simulink model "quadrotor_lqr_v3"  (R2026a)
settings: Solver=ode4  StopTime=15  FixedStep=1e-3
PreLoadFcn:
  | run('init_params.m'); if exist('controller_data.mat','file'), load('controller_data.mat'); end
values from neighbouring files (symbols this model uses):
  K = [3.16227766017 -4.72567955818e-17 -8.28019285395e-17 -1.64313429263e-16 4.90965597244 1.71076429981e-16 -5.36515533389e-17 3.94835012882e-16 5.96978589095e-16 2.2360679775 -3.44681097997e-15 8.87033425726e-16 ... (32 elements, 4x8)]    [controller_data.mat]    (also in design_lqr.m = lqr(A, B, Q, R))
undefined symbols (not defined in the file or in its folder): ic, params, ref, sat
settings Model: FPTShortcutValueString='{{},{''BaselineRun'',1,1,1,''BaselineRun'','''',{},''M'','''',''''},{''BaselineRun_2'',1,1,1,''BaselineRun_2'','''',{},''M'','''',''''}}'  Creator=yusuf  LastModifiedBy=yusuf

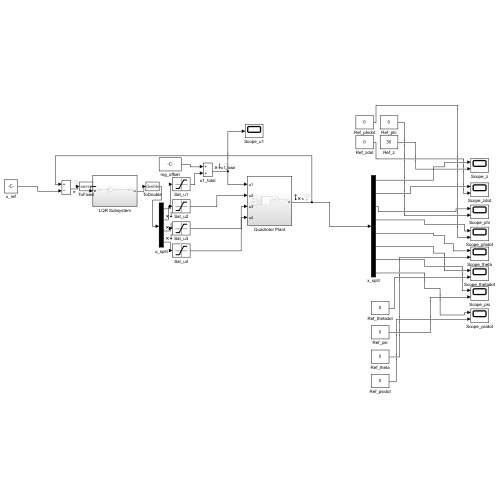
[thumbnail: Simulink's stored preview of the top-level diagram]
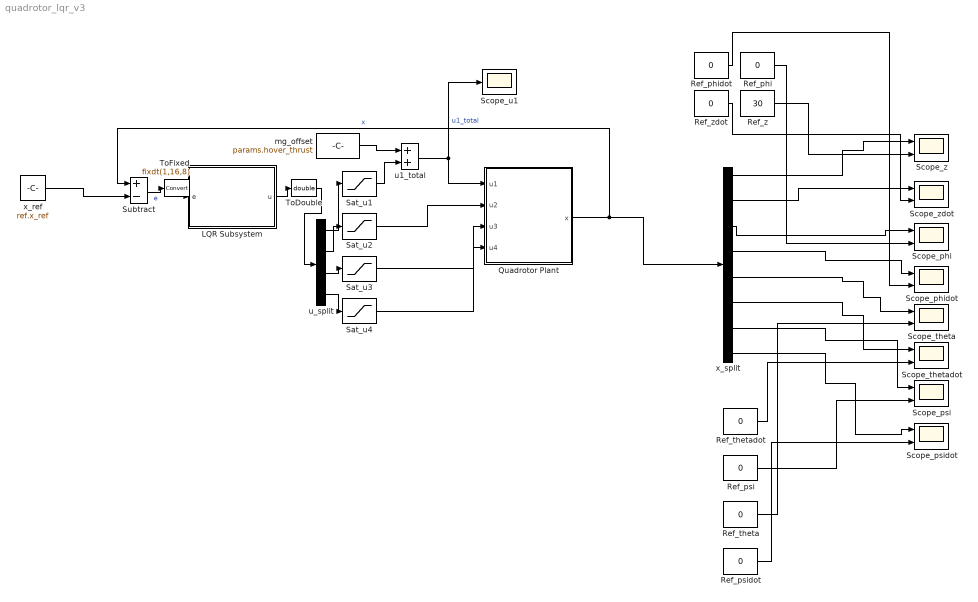
== system quadrotor_lqr_v3 ==
  LQR Subsystem : Subsystem
  Quadrotor Plant : Subsystem
  Ref_phi : Constant  Value=0  SampleTime=1e-3
  Ref_phidot : Constant  Value=0  SampleTime=1e-3
  Ref_psi : Constant  Value=0  SampleTime=1e-3
  Ref_psidot : Constant  Value=0  SampleTime=1e-3
  Ref_theta : Constant  Value=0  SampleTime=1e-3
  Ref_thetadot : Constant  Value=0  SampleTime=1e-3
  Ref_z : Constant  Value=30  SampleTime=1e-3
  Ref_zdot : Constant  Value=0  SampleTime=1e-3
  Sat_u1 : Saturate  UpperLimit=sat.u1_upper  LowerLimit=sat.u1_lower
  Sat_u2 : Saturate  UpperLimit=sat.tau_max  LowerLimit=-sat.tau_max
  Sat_u3 : Saturate  UpperLimit=sat.tau_max  LowerLimit=-sat.tau_max
  Sat_u4 : Saturate  UpperLimit=sat.tau_max  LowerLimit=-sat.tau_max
  Scope_phi : Scope  NumInputPorts=2
      settings: ActiveDisplayYMinimum=-1.8573314435984112  ActiveDisplayYMaximum=16.715982992385705  DataLoggingVariableName=ScopeData2
  Scope_phidot : Scope  NumInputPorts=2
      settings: ActiveDisplayYMinimum=-1.055862335568192  ActiveDisplayYMaximum=0.24970117270907188  DataLoggingVariableName=ScopeData3
  Scope_psi : Scope  NumInputPorts=2
      settings: ActiveDisplayYMinimum=-1.8573314435984112  ActiveDisplayYMaximum=16.715982992385705  DataLoggingVariableName=ScopeData6
  Scope_psidot : Scope  NumInputPorts=2
      settings: ActiveDisplayYMinimum=-1.8573314435984112  ActiveDisplayYMaximum=16.715982992385705  DataLoggingVariableName=ScopeData7
  Scope_theta : Scope  NumInputPorts=2
      settings: ActiveDisplayYMinimum=-1.8573314435984112  ActiveDisplayYMaximum=16.715982992385705  DataLoggingVariableName=ScopeData4
  Scope_thetadot : Scope  NumInputPorts=2
      settings: ActiveDisplayYMinimum=-1.8573314435984112  ActiveDisplayYMaximum=16.715982992385705  DataLoggingVariableName=ScopeData5
  Scope_u1 : Scope
      settings: ActiveDisplayYMinimum=-5.2464765259022688  ActiveDisplayYMaximum=24.907669578101633
  Scope_z : Scope  NumInputPorts=2
      settings: ActiveDisplayYMinimum=-3.7505255254254628  ActiveDisplayYMaximum=33.754729728829176
  Scope_zdot : Scope  NumInputPorts=2
      settings: ActiveDisplayYMinimum=-1  ActiveDisplayYMaximum=1
  Subtract : Sum  Inputs=+-  SampleTime=1e-3
  ToDouble : DataTypeConversion  OutDataTypeStr=double  SaturateOnIntegerOverflow=off  RndMeth=Floor
  ToFixed : DataTypeConversion  OutDataTypeStr=fixdt(1,16,8)  SampleTime=1e-3  SaturateOnIntegerOverflow=off  RndMeth=Floor
  mg_offset : Constant  Value=params.hover_thrust  SampleTime=1e-3
  u1_total : Sum
  u_split : Demux
  x_ref : Constant  Value=ref.x_ref  SampleTime=1e-3
  x_split : Demux  Outputs=8
  wires:
  x_ref/1 -> Subtract/2
  mg_offset/1 -> u1_total/1
  u1_total/1 -> Quadrotor Plant/1(u1), Scope_u1/1  "u1_total"
  Quadrotor Plant/1(x) -> x_split/1, Subtract/1  "x"
  Subtract/1 -> ToFixed/1  "e"
  ToFixed/1 -> LQR Subsystem/1(e)
  LQR Subsystem/1(u) -> ToDouble/1
  ToDouble/1 -> u_split/1
  u_split/1 -> Sat_u1/1
  u_split/2 -> Sat_u2/1
  u_split/3 -> Sat_u3/1
  u_split/4 -> Sat_u4/1
  Sat_u1/1 -> u1_total/2
  Sat_u2/1 -> Quadrotor Plant/2(u2)
  Sat_u3/1 -> Quadrotor Plant/3(u3)
  Sat_u4/1 -> Quadrotor Plant/4(u4)
  x_split/1 -> Scope_z/1
  x_split/2 -> Scope_zdot/1
  x_split/3 -> Scope_phi/1
  x_split/4 -> Scope_phidot/1
  x_split/5 -> Scope_theta/1
  x_split/6 -> Scope_thetadot/1
  x_split/7 -> Scope_psi/1
  x_split/8 -> Scope_psidot/1
  Ref_z/1 -> Scope_z/2
  Ref_zdot/1 -> Scope_zdot/2
  Ref_phi/1 -> Scope_phi/2
  Ref_phidot/1 -> Scope_phidot/2
  Ref_theta/1 -> Scope_theta/2
  Ref_thetadot/1 -> Scope_thetadot/2
  Ref_psi/1 -> Scope_psi/2
  Ref_psidot/1 -> Scope_psidot/2

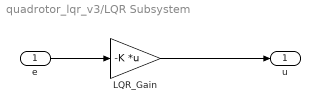
== system quadrotor_lqr_v3/LQR Subsystem ==
  e : Inport  OutDataTypeStr=fixdt(1,16,8)  SampleTime=1e-3
  LQR_Gain : Gain  Gain=-K  Multiplication=Matrix(K*u)  OutDataTypeStr=fixdt(1,16,6)
  u : Outport  OutDataTypeStr=fixdt(1,16,6)
  wires:
  e/1 -> LQR_Gain/1
  LQR_Gain/1 -> u/1

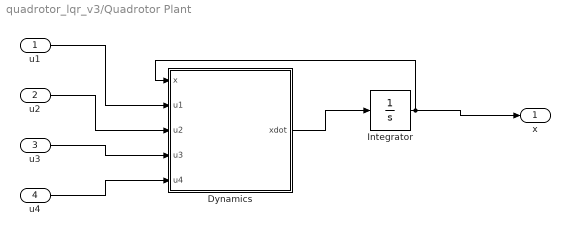
== system quadrotor_lqr_v3/Quadrotor Plant ==
  u1 : Inport
  u2 : Inport  Port=2
  u3 : Inport  Port=3
  u4 : Inport  Port=4
  Dynamics : MATLAB Function  TreatAsAtomicUnit=on
  Integrator : Integrator  InitialCondition=ic.x0
  x : Outport
  wires:
  u1/1 -> Dynamics/2(u1)
  u2/1 -> Dynamics/3(u2)
  u3/1 -> Dynamics/4(u3)
  u4/1 -> Dynamics/5(u4)
  Dynamics/1(xdot) -> Integrator/1
  Integrator/1 -> x/1, Dynamics/1(x)

== matlab function quadrotor_lqr_v3/Quadrotor Plant/Dynamics ==
  data: x input; xdot output; u1 input; u2 input; u3 input; u4 input
function xdot = dynamics(x, u1, u2, u3, u4)
% Quadrotor nonlinear dynamics - Khati et al. eq. 15
% State: x = [z, zdot, phi, phidot, theta, thetadot, psi, psidot]
% Input: u1 = thrust, u2/u3/u4 = roll/pitch/yaw torques

% Parameters (Khati Table I - hard-coded for HDL Coder compatibility)
Ix = 7.5e-3;  Iy = 7.5e-3;  Iz = 1.3e-2;
m  = 0.65;    g  = 9.81;
K1z = 6.354e-4;
K2x = 5.56e-4; K2y = 5.56e-4; K2z = 6.354e-4;

% Unpack state
zdot     = x(2);
phi      = x(3);
phidot   = x(4);
theta    = x(5);
thetadot = x(6);
psidot   = x(8);

% Translational (altitude, z-axis)
zddot = -g + (cos(phi)*cos(theta)/m)*u1 - (K1z/m)*zdot;

% Rotational (roll, pitch, yaw)
phiddot   = ((Iy - Iz)/Ix)*thetadot*psidot - (K2x/Ix)*phidot + (1/Ix)*u2;
thetaddot = ((Iz - Ix)/Iy)*phidot*psidot   - (K2y/Iy)*thetadot + (1/Iy)*u3;
psiddot   = ((Ix - Iy)/Iz)*phidot*thetadot - (K2z/Iz)*psidot   + (1/Iz)*u4;

% xdot
xdot = zeros(8,1);
xdot(1) = x(2);
xdot(2) = zddot;
xdot(3) = x(4);
xdot(4) = phiddot;
xdot(5) = x(6);
xdot(6) = thetaddot;
xdot(7) = x(8);
xdot(8) = psiddot;
end
